simulink model "ukl_reg_ciagly"  (Simulink 10.1)
settings: Solver=ode3  StartTime=0.0  StopTime=200  FixedStep=tc  RelTol=1e-3
libraries: cstblocks x2
settings Model: Creator=RafalG  LastModifiedBy=Rafal
settings DataIOCC: SignalLoggingSaveFormat=ModelDataLogs
settings OptimizationCC: ExpressionDepthLimit=2147483647
settings DebuggingCC: SolverPrmCheckMsg=warning  FcnCallInpInsideContextMsg=warning  StateNameClashWarn=warning

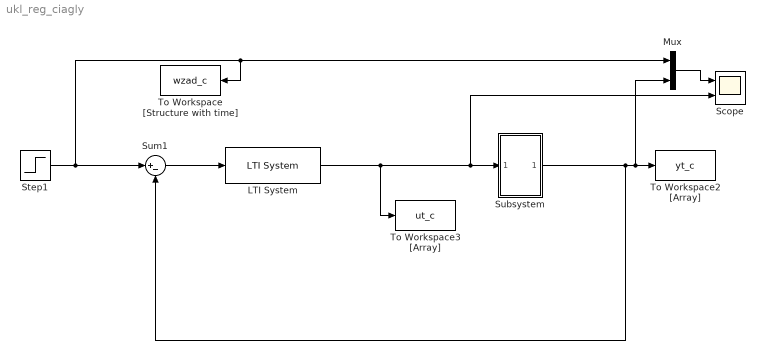
== system ukl_reg_ciagly ==
  LTI System : cstblocks/LTI System  sys=Kr  IC=[]
  Mux : Mux  Inputs=2
  Scope : Scope  NumInputPorts=2
  Step1 : Step  Time=0  SampleTime=0
  Subsystem : Subsystem
  Sum1 : Sum  Inputs=|+-
  To Workspace [Structure with time] : ToWorkspace  VariableName=wzad_c  SaveFormat=Structure With Time  SampleTime=-1
  To Workspace2 [Array] : ToWorkspace  VariableName=yt_c  SampleTime=-1
  To Workspace3 [Array] : ToWorkspace  VariableName=ut_c  SaveFormat=Timeseries  SampleTime=-1
  wires:
  Sum1/1 -> LTI System/1
  Subsystem/1(Out1) -> To Workspace2 [Array]/1, Mux/2, Sum1/2
  Mux/1 -> Scope/1
  LTI System/1 -> To Workspace3 [Array]/1, Subsystem/1(In1), Scope/2
  Step1/1 -> Sum1/1, Mux/1, To Workspace [Structure with time]/1

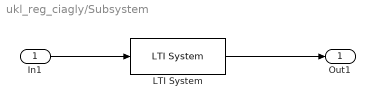
== system ukl_reg_ciagly/Subsystem ==
  In1 : Inport
  LTI System : cstblocks/LTI System  sys=K  IC=[]
  Out1 : Outport
  wires:
  In1/1 -> LTI System/1
  LTI System/1 -> Out1/1
